simulink model "Modulator_CT"  (R2025b)
settings: Solver=ode4  StartTime=0.0  StopTime=1  MaxStep=1e-8  RelTol=1e-3
model workspace (MAT data in the model file):
  Delay_80 = [0 0 0]
  ENOB_80 = 3.17460069492
  FUNDF_80 = [100.000147315 1899.80481457]
  FUNDX_80 = [25.5869777506 0.142795289221]
  IMODF_80 = [nan 3708.52309694]
  IMODX_80 = [nan -81.8171361401]
  NoiseFloor_80 = -77.867787316
  OIP3_80 = nan
  SFDR_80 = 24.8872320778
  SINAD_80 = 20.8710961834
  SNR_80 = 20.8710984866
  THD_80 = -58.2888809054
  Var1 = 0
  delay_80 = [0 0 0]
  ts = 0.0001
undefined symbols (not defined in the file or in its folder): den, dspblkCoreblockFVToolHelper, gcbh, num, Ts_mod
libraries: dspmlti4 x2, dspsigops x1
settings Model: VariantFading=off  Creator=anurag jaiswal  LastModifiedBy=divijsharma
settings DataIOCC: SaveOutput=off  SignalLogging=off  DSMLogging=off  SaveTime=off  ReturnWorkspaceOutputs=off

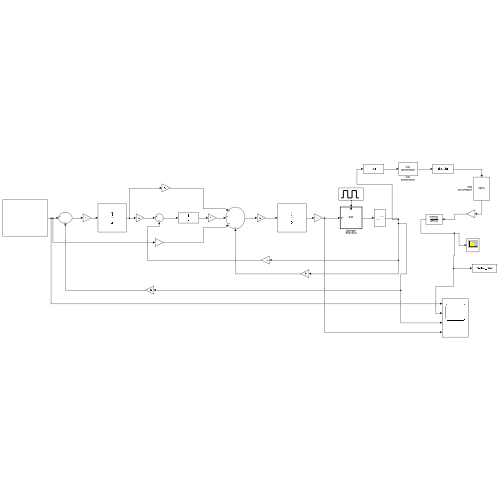
[thumbnail: Simulink's stored preview of the top-level diagram]
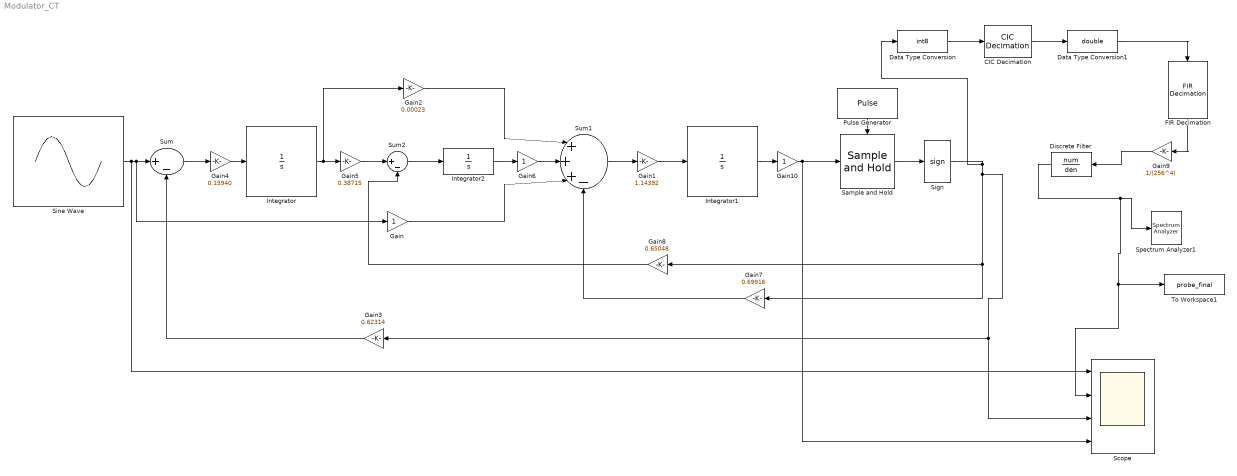
== system Modulator_CT ==
  CIC Decimation : dspmlti4/CIC Decimation  filtFrom=Dialog parameters  filtobj=CICDECIM  ftype=Decimator  R=256  M=1  N=4  filterInternals=Minimum section word lengths  BPS=[16 16 16 16]  FLPS=0  outputWordLength=32  outputFracLength=0  launchFVT=off  framing=Maintain input frame rate  RateOptions=Allow multirate processing
      settings: LibrarySourceBlock=|
      | dsphdlsupportfiltering/CIC
      | Decimation
  Data Type Conversion : DataTypeConversion  OutDataTypeStr=int8  SaturateOnIntegerOverflow=off  RndMeth=Floor
  Data Type Conversion1 : DataTypeConversion  OutDataTypeStr=double  RndMeth=Nearest  SaturateOnIntegerOverflow=off
  Discrete Filter : DiscreteFilter  LoadFcn=dspblkCoreblockFVToolHelper(gcbh,'load');  Numerator=num  Denominator=den
      settings: CopyFcn=dspblkCoreblockFVToolHelper(gcbh,'copy');  DeleteFcn=dspblkCoreblockFVToolHelper(gcbh,'close');  ModelCloseFcn=dspblkCoreblockFVToolHelper(gcbh,'close');  PreSaveFcn=dspblkCoreblockFVToolHelper(gcbh,'presave');  PostSaveFcn=dspblkCoreblockFVToolHelper(gcbh,'postsave');  CloseFcn=dspblkCoreblockFVToolHelper(gcbh,'close');
  FIR Decimation : dspmlti4/FIR Decimation  FilterSource=Dialog parameters  h=b_fir  D=2  filtStruct=Direct form  FilterObject=FDECIM  framing=Allow multirate processing  AllowArbitraryInputLength=off  inputOffset=0  outputBufInitCond=0  roundingMode=Floor  overflowMode=off  firstCoeffDataTypeStr=Inherit: Same word length as input  firstCoeffMin=[]  firstCoeffMax=[]  firstCoeffLastDataTypeStr=Inherit: Same word length as input  outputDataTypeStr=Inherit: Same as accumulator  outputMin=[]  outputMax=[]  outputLastDataTypeStr=Inherit: Same as accumulator
      settings: LibrarySourceBlock=|
      | dsphdlsupportfiltering/FIR
      | Decimation
  Gain : Gain
  Gain1 : Gain  Gain=1.14392
  Gain10 : Gain
  Gain2 : Gain  Gain=0.00023
  Gain3 : Gain  Gain=0.62314
  Gain4 : Gain  Gain=0.15940
  Gain5 : Gain  Gain=0.38715
  Gain6 : Gain
  Gain7 : Gain  Gain=0.69916
  Gain8 : Gain  Gain=0.65048
  Gain9 : Gain  Gain=1/(256^4)
  Integrator : Integrator
  Integrator1 : Integrator
  Integrator2 : Integrator
  Pulse Generator : DiscretePulseGenerator  PulseType=Time based  Period=1/(512e3)  PulseWidth=50  SampleTime=Ts_mod
  Sample and Hold : dspsigops/Sample and Hold  trig=Rising edge  initCond=0  latchinput=off
  Scope : Scope  NumInputPorts=4
      settings: ActiveDisplayYMinimum=-0.74999999999999989  ActiveDisplayYMaximum=0.74999999999999989
  Sign : Signum
  Sine Wave : Sin  Amplitude=0.6  Frequency=2*pi*100  SampleTime=0
  Spectrum Analyzer1 : SpectrumAnalyzer  WindowPosition=[1.000000,1.000000,1280.000000,741.000000,]  Visible=on  ScopeFrameLocation=window  WindowInvariantSamplesPerUpdate=on  Span=4000  StartFrequency=-2000  StopFrequency=2000  YLimits=[-67.7642 31.7308]  SelectedToolstripTab=spectrumAnalyzerToolstrip.channelMeasurementsTab
  Sum : Sum  Inputs=|+-
  Sum1 : Sum  Inputs=|+++-
  Sum2 : Sum  Inputs=|+-
  To Workspace1 : ToWorkspace  VariableName=probe_final  SampleTime=-1
      settings: Save2DSignal=2-D array (concatenate along first dimension)
  wires:
  Sine Wave/1 -> Scope/1, Gain/1, Sum/1
  Pulse Generator/1 -> Sample and Hold/Trigger
  Integrator/1 -> Gain2/1, Gain5/1
  Integrator2/1 -> Gain6/1
  Sum/1 -> Gain4/1
  Sample and Hold/1 -> Sign/1
  Gain3/1 -> Sum/2
  Gain4/1 -> Integrator/1
  Gain6/1 -> Sum1/2
  Gain1/1 -> Integrator1/1
  Sum1/1 -> Gain1/1
  Integrator1/1 -> Gain10/1
  Gain/1 -> Sum1/3
  Gain2/1 -> Sum1/1
  Gain7/1 -> Sum1/4
  Gain5/1 -> Sum2/1
  Sum2/1 -> Integrator2/1
  Gain8/1 -> Sum2/2
  CIC Decimation/1 -> Data Type Conversion1/1
  Data Type Conversion/1 -> CIC Decimation/1
  Sign/1 -> Data Type Conversion/1, Gain7/1, Gain8/1, Gain3/1, Scope/3
  Gain10/1 -> Scope/4, Sample and Hold/1
  Data Type Conversion1/1 -> FIR Decimation/1
  Gain9/1 -> Discrete Filter/1
  Discrete Filter/1 -> Scope/2, To Workspace1/1, Spectrum Analyzer1/1
  FIR Decimation/1 -> Gain9/1
